simulink model "uacs_plant_ref"  (R2024a)
settings: Solver=ode4  StartTime=0.0  StopTime=sim_t_end  FixedStep=sim_ts_ctrl  RelTol=1e-3
undefined symbols (not defined in the file): ref_h_from_state, ref_h_isa, ref_inertia, ref_mass
libraries: aerolibprivatev1p5 x1, aerolibatmos2 x1
settings Model: Creator=Ash Trailer  LastModifiedBy=Ash Trailer
settings DataIOCC: SaveFormat=StructureWithTime
settings DebuggingCC: AlgebraicLoopMsg=error

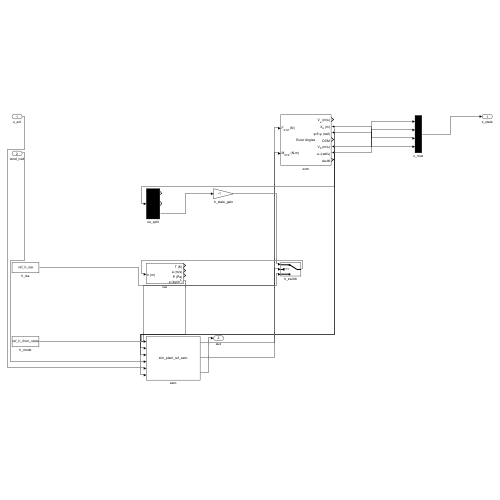
[thumbnail: Simulink's stored preview of the top-level diagram]
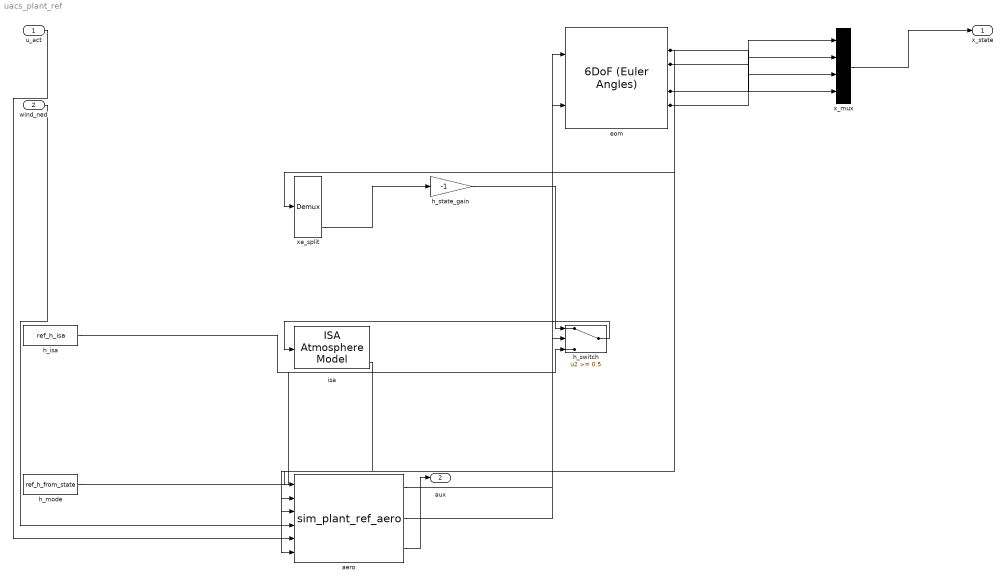
== system uacs_plant_ref ==
  u_act : Inport
  wind_ned : Inport  Port=2
  aero : M-S-Function  FunctionName=sim_plant_ref_aero
  eom : aerolibprivatev1p5/6DoF (Euler Angles)  xme_0=ref_x0_pos  Vm_0=ref_x0_vb  eul_0=ref_x0_eul  pm_0=ref_x0_om  Mass=ref_mass  Inertia=ref_inertia
  h_isa : Constant  Value=ref_h_isa
  h_mode : Constant  Value=ref_h_from_state
  h_state_gain : Gain  Gain=-1
  h_switch : Switch  Threshold=0.5  SaturateOnIntegerOverflow=off  InputSameDT=off
  isa : aerolibatmos2/ISA Atmosphere Model  useExtended=off  action=Warning  custom=off  viscosityOut=off  g=9.80665  gamma=1.4  R=287.0531  L=0.0065  h_trop=11000  h_strat=20000  rho0=1.225  P0=101325  T0=288.15  h0=0  S=110.4  Tref=273.15  muref=1.716e-5
  x_mux : Mux
  xe_split : Demux  Outputs=3
  x_state : Outport
  aux : Outport  Port=2
  wires:
  h_switch/1 -> isa/1
  h_isa/1 -> h_switch/3
  h_mode/1 -> h_switch/2
  eom/2 -> xe_split/1, x_mux/4
  xe_split/3 -> h_state_gain/1
  h_state_gain/1 -> h_switch/1
  eom/5 -> aero/1, x_mux/1
  eom/6 -> aero/2, x_mux/2
  eom/3 -> aero/3, x_mux/3
  wind_ned/1 -> aero/4
  u_act/1 -> aero/5
  isa/4 -> aero/6
  aero/1 -> eom/1
  aero/2 -> eom/2
  x_mux/1 -> x_state/1
  aero/3 -> aux/1
